simulink model "sl_drivepose"  (R2019b)
settings: Solver=ode45  StartTime=0.0  StopTime=20.0  MaxStep=0.05  RelTol=1e-3  EnableMultiTasking=on
InitFcn:
  | if exist('x0')
  |   assert(length(x0) == 3, 'x0 must be a 3-vector');
  | else
  |   x0 = [9 5 0];
  |   msgbox(sprintf('x0 not defined in workspace, setting it to [%g %g %g]\n', x0));
  | end
  | if exist('xg')
  |   assert(length(xg) == 3, 'xg must be a 3-vector');
  | else
  |   xg = [5 5 pi/2];
  |   msgbox(sprintf('xg not defined in workspace, setting it to [%g %g %g]\n', xg));
  | end
  | % clean up old vehicle icons
  | set(0, 'ShowHiddenHandles', 'on')
  | delete(findobj('Tag', 'vehicle'))
  | set(0, 'ShowHiddenHandles', 'off')
StopFcn:
  | % update the XY scope
  | set(0, 'ShowHiddenHandles', 'on')
  | fig = findobj('name', 'XY');
  | ax = findobj(fig, 'type', 'axes');
  | axes(ax)
  | grid on
  | hold on
  | plot_vehicle(x0, 'r', 'Tag', 'vehicle')
  | plot_vehicle(xg, 'b', 'Tag', 'vehicle')
  | hold off
  | set(0, 'ShowHiddenHandles', 'off')
libraries: simulink x2, roblocks x1
settings Model: Creator=pic  LastModifiedBy=corkep
settings DataIOCC: SaveFormat=Array  SaveState=on  TimeSaveName=t  OutputSaveName=y
settings OptimizationCC: ExpressionDepthLimit=2147483647  LifeSpan=inf
settings DebuggingCC: UnderspecifiedInitializationDetection=Classic  MergeDetectMultiDrivingBlocksExec=none  SolverPrmCheckMsg=warning  AllowSymbolicDim=off  StateNameClashWarn=warning  PregeneratedLibrarySubsystemCodeDiagnostic=none  SFUnexpectedBacktrackingDiag=warning  SFNoUnconditionalDefaultTransitionDiag=warning  SFExecutionAtInitializationDiag=none  ArithmeticOperatorsInVariantConditions=warning
settings HardwareCC: ProdBitPerPointer=32  ProdBitPerSizeT=32  ProdBitPerPtrDiffT=32  ProdLargestAtomicFloat=None  ProdIntDivRoundTo=Undefined  ProdEndianess=Unspecified  ProdWordSize=32  ProdHWDeviceType=32-bit Generic
settings ModelReferenceCC: PropagateSignalLabelsOutOfModel=off
settings SFSimCC: SimUseLocalCustomCode=off  CustomCodeUndefinedFunction=UseInterfaceOnly
settings RTWCC: RTWUseLocalCustomCode=off
settings CodeAppCC: StateflowObjectComments=on
settings GRTTargetCC: TargetLangStandard=C89/C90 (ANSI)  GeneratePreprocessorConditionals=Disable all  CombineOutputUpdateFcns=off  GRTInterface=on
settings ConfigComp: CovMetricSettings=dw  CovHtmlReporting=on  CovSaveCumulativeToWorkspaceVar=on  CovSaveSingleToWorkspaceVar=on  CovExternalEMLEnable=off

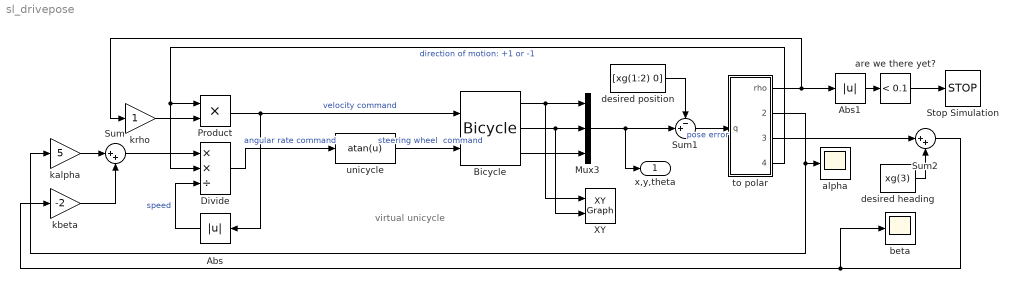
== system sl_drivepose ==
  note: virtual unicycle
  Abs : Abs
  Abs1 : Abs
  Bicycle : roblocks/Vehicles/Bicycle  vlim=1  accel=1  alim=1  steer_rate=Inf  L=1  x0=x0
  Divide : Product  Inputs=**/
  Mux3 : Mux  Inputs=3
  Product : Product  RndMeth=Zero
  Stop Simulation : Stop
  Sum : Sum  Inputs=|++
  Sum1 : Sum  Inputs=-+|
  Sum2 : Sum  Inputs=|++
  XY : simulink/Sinks/XY Graph  xmin=0  xmax=10  ymin=0  ymax=10  st=-1
  alpha : Scope
  are we there yet? : simulink/Logic and Bit Operations/Compare To Constant  relop=<  const=0.1  OutDataTypeStr=boolean
  beta : Scope
  desired heading : Constant  Value=xg(3)
  desired position : Constant  Value=[xg(1:2) 0]
  kalpha : Gain  Gain=5
  kbeta : Gain  Gain=-2
  krho : Gain
  to polar : Subsystem
  "unicycle " : Fcn  Expr=atan(u)
  x,y,theta : Outport  VectorParamsAs1DForOutWhenUnconnected=off
  wires:
  Mux3/1 -> x,y,theta/1, Sum1/2
  Bicycle/1 -> Mux3/1, XY/1
  Bicycle/2 -> Mux3/2, XY/2
  Bicycle/3 -> Mux3/3
  to polar/2(alpha) -> kalpha/1, alpha/1
  kalpha/1 -> Sum/1
  kbeta/1 -> Sum/2
  Product/1 -> Bicycle/1, Abs/1  "velocity command"
  krho/1 -> Product/2
  to polar/1(rho) -> Abs1/1, krho/1
  to polar/4(direction) -> Product/1, Divide/2  "direction of motion: +1 or -1"
  desired position/1 -> Sum1/1
  Sum1/1 -> to polar/1(q)  "pose error"
  Sum/1 -> Divide/1
  are we there yet?/1 -> Stop Simulation/1
  to polar/3(beta) -> Sum2/1
  Sum2/1 -> kbeta/1, beta/1
  desired heading/1 -> Sum2/2
  Divide/1 -> "unicycle "/1  "angular rate command"
  Abs/1 -> Divide/3  "speed"
  "unicycle "/1 -> Bicycle/2  "steering wheel  command"
  Abs1/1 -> are we there yet?/1

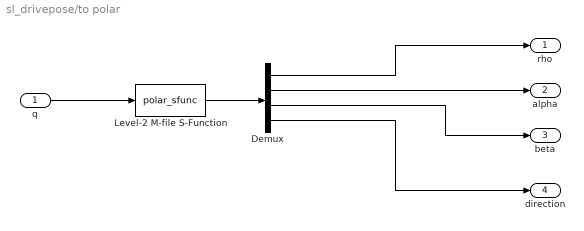
== system sl_drivepose/to polar ==
  q : Inport
  Demux : Demux
  Level-2 M-file S-Function : M-S-Function  FunctionName=polar_sfunc
  rho : Outport  VectorParamsAs1DForOutWhenUnconnected=off
  alpha : Outport  Port=2  VectorParamsAs1DForOutWhenUnconnected=off
  beta : Outport  Port=3  VectorParamsAs1DForOutWhenUnconnected=off
  direction : Outport  Port=4  VectorParamsAs1DForOutWhenUnconnected=off
  wires:
  Demux/3 -> beta/1
  q/1 -> Level-2 M-file S-Function/1
  Level-2 M-file S-Function/1 -> Demux/1
  Demux/1 -> rho/1
  Demux/2 -> alpha/1
  Demux/4 -> direction/1
